simulink model "MPPT_PI_p&o PartIALShading"  (R2024b)
settings: Solver=VariableStepAuto  StartTime=0.0  StopTime=1  FixedStep=1e-6  RelTol=1e-4
libraries: spsDiodeLib x5, spsPVArrayLib x4, spsSeriesRLCBranchLib x4, spsVoltageMeasurementLib x3, spsCurrentMeasurementLib x2, spsMosfetLib x1, slpidlib x1, simulink x1, sps_lib x1
settings Model: Creator=VICTUS  LastModifiedBy=VICTUS
settings SolverCC: ZeroCrossAlgorithm=Adaptive
settings DebuggingCC: MaskedZcDiagnostic=none  IgnoredZcDiagnostic=none

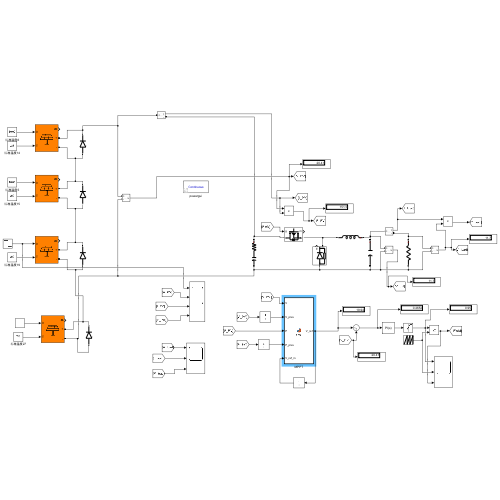
[thumbnail: Simulink's stored preview of the top-level diagram]
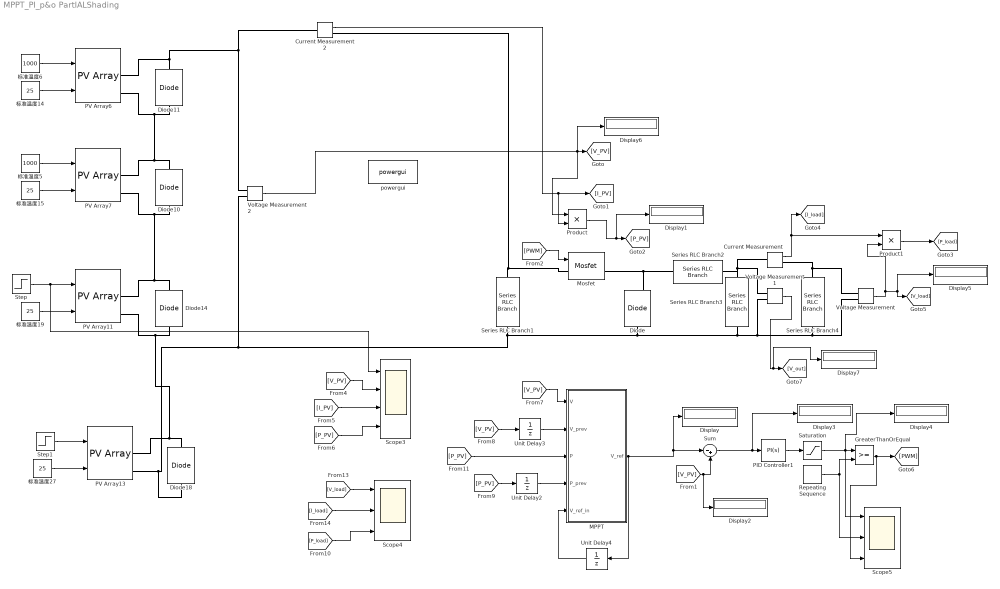
== system MPPT_PI_p&o PartIALShading ==
  Current Measurement : spsCurrentMeasurementLib/Current Measurement  PhasorSimulation=off  OutputType=Complex  PSBequivalent=0
  Current Measurement2 : spsCurrentMeasurementLib/Current Measurement  PhasorSimulation=off  OutputType=Complex  PSBequivalent=0
  Diode : spsDiodeLib/Diode  Ron=0.001  Lon=0  Vf=0.8  IC=0  UseSnubber=0  Rs=500  Cs=250e-9  Measurements=on
  Diode{10..11,14,18} (4 alike) : spsDiodeLib/Diode  Ron=0.001  Lon=0  Vf=0.8  IC=0  UseSnubber=off  Rs=inf  Cs=250e-9  Measurements=off
  Display{,1..7} (8 alike) : Display
  GreaterThanOrEqual : RelationalOperator  OutDataTypeStr=boolean  RndMeth=Simplest  InputSameDT=off
  MPPT : MATLAB Function  TreatAsAtomicUnit=on
  Mosfet : spsMosfetLib/Mosfet  Ron=0.1  Lon=0  Rd=0.01  Vfd=0  IC=0  Rs=1e5  Cs=inf  Measurements=on
  PID Controller1 : slpidlib/PID Controller  Controller=PI  Form=Parallel  TimeDomain=Continuous-time  UseExternalTs=off  SampleTime=-1  IntegratorMethod=Forward Euler  FilterMethod=Forward Euler  ControllerParametersSource=internal  P=1  I=1  UseKiTs=off  D=0  UseExternalDerivativeSource=off  N=100  UseFilter=on  TunerSelectOption=Transfer Function Based (PID Tuner App)  InitialConditionSource=internal  InitialConditionForIntegrator=0  InitialConditionForFilter=0  DifferentiatorICPrevScaledInput=0  ExternalReset=none  TrackingMode=off  Kt=1  LimitOutput=off  SatLimitsSource=internal  UpperSaturationLimit=inf  LowerSaturationLimit=-inf  LinearizeAsGain=on  AntiWindupMode=none  Kb=1  LimitIntegrator=off  UpperIntegratorSaturationLimit=inf  LowerIntegratorSaturationLimit=-inf  POutMin=[]  POutMax=[]  IOutMin=[]  IOutMax=[]  DOutMin=[]  DOutMax=[]  NOutMin=[]  NOutMax=[]  SumOutMin=[]  SumOutMax=[]  SaturationOutMin=[]  SaturationOutMax=[]  PParamMin=[]  PParamMax=[]  IParamMin=[]  IParamMax=[]  DParamMin=[]  DParamMax=[]  NParamMin=[]  NParamMax=[]  KbParamMin=[]  KbParamMax=[]  KtParamMin=[]  KtParamMax=[]  KbOutMin=[]  KbOutMax=[]  KtOutMin=[]  KtOutMax=[]  IntegratorOutMin=[]  IntegratorOutMax=[]  FilterOutMin=[]  FilterOutMax=[]  SumI1OutMin=[]  SumI1OutMax=[]  SumI2OutMin=[]  SumI2OutMax=[]  SumI3OutMin=[]  SumI3OutMax=[]  SumI4OutMin=[]  SumI4OutMax=[]  SumDOutMin=[]  SumDOutMax=[]  DifferentiatorOutMin=[]  DifferentiatorOutMax=[]  FilterDiffOutCoefMin=[]  FilterDiffOutCoefMax=[]  ReciprocalOutMin=[]  ReciprocalOutMax=[]  SumDenOutMin=[]  SumDenOutMax=[]  SumNumOutMin=[]  SumNumOutMax=[]  DivideOutMin=[]  DivideOutMax=[]  UdiffTsProdOutMin=[]  UdiffTsProdOutMax=[]  NTsProdOutMin=[]  NTsProdOutMax=[]  UintegralTsProdOutMin=[]  UintegralTsProdOutMax=[]  UngainTsProdOutMin=[]  UngainTsProdOutMax=[]  ClampingZeroOutDataTypeStr=Inherit: Inherit via back propagation  ClampingZeroOutMin=[]  ClampingZeroOutMax=[]  FilterDenConstantOutDataTypeStr=Inherit: Inherit via back propagation  FilterDenConstantOutMin=[]  FilterDenConstantOutMax=[]  PCopyOutDataTypeStr=Inherit: Inherit via back propagation  PCopyOutMin=[]  PCopyOutMax=[]  NCopyOutDataTypeStr=Inherit: Inherit via back propagation  NCopyOutMin=[]  NCopyOutMax=[]  IntegratorContinuousStateAttributes=''  IntegratorStateMustResolveToSignalObject=off  IntegratorRTWStateStorageClass=Auto  FilterContinuousStateAttributes=''  FilterStateMustResolveToSignalObject=off  FilterRTWStateStorageClass=Auto  ParallelPVariant=InternalParameters  IdealPVariant=Disabled  IVariant=InternalParameters  DVariant=Disabled  IntegratorVariant=Continuous  SatVariant=Disabled  AWVariant=Passthrough  PCopyVariant=Disabled  TRVariant=Disabled  FdbkBlocksVariant=Forward  IdealPFdbkVariant=Disabled  SatFdbkVariant=Disabled  DerivativeFilterVariant=Disabled  NVariant=Disabled  NCopyVariant=Disabled_SignalSpec  FilterICVariant=Disabled  IntegratorICVariant=InternalICs  ExternalResetVariant=Disabled  TRSumVariant=Passthrough  SumFdbkVariant=Disabled  SumVariant=Sum_PI  TsampFilterVariant=InternalTs  TsampNgainVariant=Passthrough  TsampIntegralVariant=Disabled_SignalSpec  ExternalSaturationOutDataTypeStr=Inherit: Same as second input  DerivativeSourceVariant=Disabled  PreIntVariant=InternalPreInt
  PV Array{6..7,11,13} (4 alike) : spsPVArrayLib/PV Array  Npar=1  Nser=1  PlotType=array @ 1000 W/m2 & specified temperatures  S_vec="[ 1000  500  100 ]"  Temp_C_vec="[ 45 25  ]"  ModuleName=User-defined  PlotWhenSelected=off  Pm=120.75  Ncell=16  Voc=22  Isc=7.5  Vm=17.5  Im=6.9  beta_Voc_pc=-0.36099  alpha_Isc_pc=0.102  beta_Voc=-0.079418  alpha_Isc=0.00765  IL=7.6829  I0=2.1898e-10  nI=2.2089  Rsh=50.0358  Rs=0.26399  RobustModel=off  RobustCellTemperature=313.3991  BAL=off  Tc=1e-6  Tfilter=5e-5
  Product : Product
  Product1 : Product
  Repeating Sequence : simulink/Sources/Repeating Sequence  rep_seq_t=[0 2e-4]  rep_seq_y=[0 1]
  Saturation : Saturate  UpperLimit=0.95  LowerLimit=0.05
  Scope3 : Scope  NumInputPorts=4
  Scope4 : Scope  NumInputPorts=3
  Scope5 : Scope  NumInputPorts=3
  Series RLC Branch1 : spsSeriesRLCBranchLib/Series RLC Branch  LConnTagsString=__new0  RConnTagsString=__new0  BranchType=RC  Resistance=0.001  Inductance=1e-3  SetiL0=off  InitialCurrent=0  Capacitance=1000e-6  Setx0=off  InitialVoltage=0  Measurements=None
  Series RLC Branch2 : spsSeriesRLCBranchLib/Series RLC Branch  LConnTagsString=__new0  RConnTagsString=__new0  BranchType=L  Resistance=0.001  Inductance=10e-3  SetiL0=off  InitialCurrent=0  Capacitance=1000e-6  Setx0=off  InitialVoltage=0  Measurements=None
  Series RLC Branch3 : spsSeriesRLCBranchLib/Series RLC Branch  LConnTagsString=__new0  RConnTagsString=__new0  BranchType=C  Resistance=0.001  Inductance=1e-3  SetiL0=off  InitialCurrent=0  Capacitance=300e-6  Setx0=off  InitialVoltage=0  Measurements=None
  Series RLC Branch4 : spsSeriesRLCBranchLib/Series RLC Branch  LConnTagsString=__new0  RConnTagsString=__new0  BranchType=R  Resistance=1  Inductance=1e-3  SetiL0=off  InitialCurrent=0  Capacitance=1000e-6  Setx0=off  InitialVoltage=0  Measurements=None
  Step : Step  Time=0.5  Before=1000  After=0  SampleTime=0
  Step1 : Step  Time=0.5  Before=1000  After=0  SampleTime=0
  Sum : Sum  Inputs=|-+
  Unit Delay2 : UnitDelay  SampleTime=-1  HasFrameUpgradeWarning=on
  Unit Delay3 : UnitDelay  SampleTime=-1  HasFrameUpgradeWarning=on
  Unit Delay4 : UnitDelay  InitialCondition=1  SampleTime=-1  HasFrameUpgradeWarning=on
  Voltage Measurement : spsVoltageMeasurementLib/Voltage Measurement  PhasorSimulation=off  OutputType=Complex  PSBequivalent=0
  Voltage Measurement1 : spsVoltageMeasurementLib/Voltage Measurement  PhasorSimulation=off  OutputType=Complex  PSBequivalent=0
  Voltage Measurement2 : spsVoltageMeasurementLib/Voltage Measurement  PhasorSimulation=off  OutputType=Complex  PSBequivalent=0
  powergui : sps_lib/powergui  Priority=1  SimulationMode=Continuous  SampleTime=50e-6  frequency=60  Iterations=50  frequencyindice=0  Pbase=100e6  ErrMax=1e-4  UnitsV=kV  UnitsW=MW  buscounter=0  FunctionMessages=off  echomessages=off  EnableUseOfTLC=off  CurrentSourceSwitches=off  DisableSnubberDevices=off  DisableRonSwitches=off  DisableVfSwitches=off  DisplayEquations=off  AutomaticDiscreteSolvers=off  SolverType=Tustin/Backward Euler (TBE)  Interpol=off  ExternalGateDelay=off  methode=off  Ts=100  x0status=blocks  SPID=on  SwTol=0  HookPort=off  NonlinearTolerance=1e-4  nMaxIteration=100  ContinueOnMaxIteration=off  RestoreLinks=warning  ResistiveCurrentMeasurement=off  Frange=[0:2:500]  Ylog=off  Xlog=on  ShowGrid=off  save=off  variable=ZData  structure=0  ZoomFFT=off  StartTime=0.0  cycles=1  DisplayStyle=1  fundamental=60  FreqAxis=off  MaxFrequency=1000  frequencyindicesteady=1  RmsSteady=1  display=off
  标准温度{14..15,19,27} (4 alike) : Constant  Value=25  SampleTime=0.001
  标准温度5 : Constant  Value=1000  SampleTime=0.001
  标准温度6 : Constant  Value=1000  SampleTime=0.001
  wires:
  标准温度5/1 -> PV Array7/1
  [V_load] -> Scope4/1
  [PWM] -> Mosfet/1
  Product1/1 -> [P_load]
  [I_PV] -> Scope3/3
  Voltage Measurement2/1 -> Product/1, Display6/1, [V_PV]
  标准温度14/1 -> PV Array6/2
  Voltage Measurement/1 -> Product1/2, Display5/1, [V_load]
  [I_load] -> Scope4/2
  标准温度27/1 -> PV Array13/2
  Current Measurement/1 -> [I_load], Product1/1
  Current Measurement2/1 -> Product/2, [I_PV]
  标准温度15/1 -> PV Array7/2
  标准温度6/1 -> PV Array6/1
  [P_load] -> Scope4/3
  Step/1 -> Scope3/1, PV Array11/1
  Product/1 -> Display1/1, [P_PV]
  标准温度19/1 -> PV Array11/2
  [V_PV] -> Scope3/2
  Voltage Measurement1/1 -> Display7/1, [V_out]
  [P_PV] -> Scope3/4
  Step1/1 -> PV Array13/1
  [V_PV] -> Display2/1, Sum/2
  GreaterThanOrEqual/1 -> Scope5/3, [PWM]
  Unit Delay3/1 -> MPPT/2(V_prev)
  Sum/1 -> PID Controller1/1, Display3/1
  [P_PV] -> Unit Delay2/1
  Repeating Sequence/1 -> Scope5/2, GreaterThanOrEqual/2
  [V_PV] -> MPPT/1(V)
  [P_PV] -> MPPT/3(P)
  PID Controller1/1 -> Saturation/1
  Saturation/1 -> Scope5/1, GreaterThanOrEqual/1, Display4/1
  MPPT/1(V_ref) -> Unit Delay4/1, Display/1, Sum/1
  Unit Delay4/1 -> MPPT/5(V_ref_in)
  [V_PV] -> Unit Delay3/1
  Unit Delay2/1 -> MPPT/4(P_prev)
  connections:
  Voltage Measurement2/LConn1 -- PV Array6/RConn1 -- Diode11/RConn1 -- Current Measurement2/LConn1
  Voltage Measurement/LConn1 -- Series RLC Branch4/LConn1 -- Current Measurement/RConn1
  PV Array7/RConn2 -- Diode14/RConn1 -- PV Array11/RConn1 -- Diode10/LConn1
  Series RLC Branch2/RConn1 -- Diode/RConn1 -- Mosfet/RConn1
  Series RLC Branch3/LConn1 -- Current Measurement/LConn1 -- Series RLC Branch2/LConn1 -- Voltage Measurement1/LConn1
  Series RLC Branch4/RConn1 -- Series RLC Branch3/RConn1 -- Voltage Measurement2/LConn2 -- PV Array13/RConn2 -- Diode18/LConn1 -- Series RLC Branch1/RConn1 -- Diode/LConn1 -- Voltage Measurement1/LConn2 -- Voltage Measurement/LConn2
  Mosfet/LConn1 -- Series RLC Branch1/LConn1 -- Current Measurement2/RConn1
  PV Array11/RConn2 -- Diode14/LConn1 -- PV Array13/RConn1 -- Diode18/RConn1
  PV Array7/RConn1 -- PV Array6/RConn2 -- Diode11/LConn1 -- Diode10/RConn1

== matlab function MPPT_PI_p&o PartIALShading/MPPT ==
  data: V input; V_ref output; V_prev input; P input; P_prev input; V_ref_in input
function V_ref = fcn(V, V_prev, P, P_prev, V_ref_in)

    step = 0.1; 

    if(P>P_prev)
        if(V>V_prev)
            V_ref = V_ref_in + step; 
        else
            V_ref = V_ref_in - step; 
        end
    else
        if(V>V_prev)
            V_ref = V_ref_in - step; 
        else
            V_ref = V_ref_in + step; 
        end
    end
    
    if(V_ref>70)
        V_ref = 70; 
    end
    if(V_ref<10)
        V_ref = 10; 
    end
